simulink model "AFC_FFNN_trainlm_45_45_45_Nor_July_15_Rep"  (R2021a)
settings: Solver=ode15s  StartTime=0.0  StopTime=T  MaxStep=.01  RelTol=1e-3
undefined symbols (not defined in the file): AF_sensor_tol, fault_time, fuel_inj_tol, kappa_tol, MAF_sensor_tol, pump_tol, tau_ww_tol, Ts, x_gain, x_offset, y_gain, y_offset
libraries: neural x140, dspsrcs4 x3
(part 4 of 6)

== system AFC_FFNN_trainlm_45_45_45_Nor_July_15_Rep/Air Fuel Control Model 1/Feed-Forward Neural Network/Layer 3/Delays 1 ==
  "p{3}" : Inport  PortDimensions=45
      mask Display: e = 0.06;c1 = [120 230 180]/255;c2 = ([120 230 180]+0)/(256+128);c3 = ([120 230 180]+128)/(256+128);patch([0 1 1 0],[0 0 1 1],c1);patch([0 1 1 1-e 1-e 0+e],[0 0 1 1-e 0+e 0+e],c2);patch([0 0 1 1-e 0+e 0+e],[0 1 1 1-e 1-e 0+e],c3);plot([0 1 1 0 0],[0 0 1 1 0]);
  mux : Mux  Inputs=1
      mask Display: e = 0.06;c1 = [120 150 230]/255;c2 = ([120 150 230]+0)/383;c3 = ([120 150 230]+128)/383;patch([0 1 1 0],[0 0 1 1],c1);patch([0 1 1 1-e 1-e 0+e],[0 0 1 1-e 0+e 0+e],c2);patch([0 0 1 1-e 0+e 0+e],[0 1 1 1-e 1-e 0+e],c3);plot([0 1 1 0 0],[0 0 1 1 0]);disp('Mux')
  "pd{3,2}" : Outport
      mask Display: e = 0.06;c1 = [120 230 180]/255;c2 = ([120 230 180]+0)/(256+128);c3 = ([120 230 180]+128)/(256+128);patch([0 1 1 0],[0 0 1 1],c1);patch([0 1 1 1-e 1-e 0+e],[0 0 1 1-e 0+e 0+e],c2);patch([0 0 1 1-e 0+e 0+e],[0 1 1 1-e 1-e 0+e],c3);plot([0 1 1 0 0],[0 0 1 1 0]);
  wires:
  mux/1 -> "pd{3,2}"/1
  "p{3}"/1 -> mux/1
